simulink model "SCDalgo_liuqenn"  (R2019a)
settings: Solver=VariableStepAuto  StartTime=0.0  StopTime=10.0  RelTol=1e-3
undefined symbols (not defined in the file or in its folder): SCDalgo_liuqenn_fp, SCDalgo_liuqenn_tp
settings Model: DataDictionary=SCDalgo_liuqenn.sldd  Creator=grandin  LastModifiedBy=mgubu

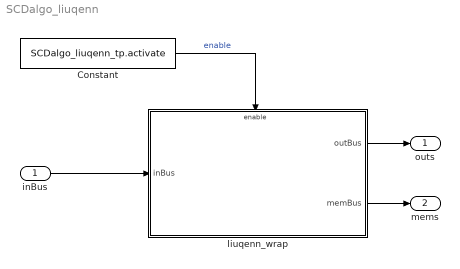
== system SCDalgo_liuqenn ==
  inBus : Inport  OutDataTypeStr=Bus: SCDalgo_liuqenn_inBus
  Constant : Constant  Value=SCDalgo_liuqenn_tp.activate
  liuqenn_wrap : Subsystem
  outs : Outport  SignalName=outBus  OutDataTypeStr=Bus: SCDalgo_liuqenn_outBus  VectorParamsAs1DForOutWhenUnconnected=on
  mems : Outport  Port=2  SignalName=memBus  OutDataTypeStr=Bus: SCDalgo_liuqenn_memBus  VectorParamsAs1DForOutWhenUnconnected=on
  wires:
  liuqenn_wrap/1(outBus) -> outs/1
  liuqenn_wrap/2(memBus) -> mems/1
  inBus/1 -> liuqenn_wrap/1(inBus)
  Constant/1 -> liuqenn_wrap/Enable  "enable"

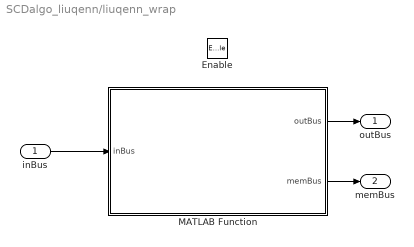
== system SCDalgo_liuqenn/liuqenn_wrap ==
  inBus : Inport
  Enable : EnablePort
  MATLAB Function : MATLAB Function  TreatAsAtomicUnit=on  SystemSampleTime=SCDalgo_liuqenn_fp.dt
  outBus : Outport  OutDataTypeStr=Bus: SCDalgo_liuqenn_outBus
  memBus : Outport  Port=2  OutDataTypeStr=Bus: SCDalgo_liuqenn_memBus
  wires:
  MATLAB Function/1(outBus) -> outBus/1
  MATLAB Function/2(memBus) -> memBus/1
  inBus/1 -> MATLAB Function/1(inBus)

== matlab function SCDalgo_liuqenn/liuqenn_wrap/MATLAB Function ==
  data: inBus input; outBus output Bus: SCDalgo_liuqenn_outBus; memBus output Bus: SCDalgo_liuqenn_memBus; SCDalgo_liuqenn_fp parameter; SCDalgo_liuqenn_tp parameter
function [outBus, memBus] = liuqenn(inBus, SCDalgo_liuqenn_fp,SCDalgo_liuqenn_tp)
% inBus: [Bm, Ff, Ia, Ip, Ft, Iu, rBt, rn, zn]
% outBus: [Fxn, Brn, Bzn]
% memBus: [=outBus]

% addtional inputs: 
%  - fixed params = SCDalgo_liuqenn_fp
%  - tunable params = SCDalgo_liuqenn_tp

FP = SCDalgo_liuqenn_fp; % fixed parameters
TP = SCDalgo_liuqenn_tp; % tunable parameters
rn = inBus.rn; zn = inBus.zn; % (r,z) coordinates
t = inBus.t;
if t >= TP.ton && t <= TP.toff % activate
    % unpack inputs
    Bm=inBus.Bm; Ff=inBus.Ff; Ia=inBus.Ia; Uf=inBus.Uf; rBt=inBus.rBt; % liuqe-rt input
    % run network inference [BM, FF, IA, UF, RBT]
    phys = [Bm;Ff;Ia;Uf;rBt];
    % [Fxn,Brn,Bzn] = liuqenn_inference_mex(phys',rn',zn');
    [Fxn,Brn,Bzn] = liuqenn_inference(phys',rn',zn');
   % fix dimensions
    Fxn = Fxn'; Brn = Brn'; Bzn=Bzn';
else % deactivated: outputs are zero everywhere
    Fxn = rn*0;
    Brn = rn*0;
    Bzn = rn*0;
end

% assign outputs
outBus.Fxn = Fxn; outBus.Brn = Brn; outBus.Bzn = Bzn;
memBus.Fxn = Fxn; memBus.Brn = Brn; memBus.Bzn = Bzn;
end
